simulink model "ecan2essai"  (Simulink 7.0)
settings: Solver=FixedStepDiscrete  StartTime=0.0  StopTime=10.0  FixedStep=0.001  RelTol=1e-3
undefined symbols (not defined in the file or in its folder): Configuration, Initialization, QEIInit, u1, u2, u3
libraries: dsPICdrivers x12, simulink x6
settings Model: Creator=Administrator  LastModifiedBy=Administrator
settings OptimizationCC: OptimizeModelRefInitCode=on  LifeSpan=1
settings DebuggingCC: SignalResolutionControl=TryResolveAllWithWarning
settings HardwareCC: ProdBitPerInt=16  ProdEndianess=LittleEndian  ProdWordSize=16  ProdHWDeviceType=16-bit Generic  TargetHWDeviceType=32-bit Generic
settings RTWCC: SystemTargetFile=dspic.tlc  TemplateMakefile=dspic_pic30_gcc.tmf  PostCodeGenCommand=dsPIC_Compile()  Description=Embedded Target for Microchip dsPIC (real-time)  GenerateReport=on  ProcessScript=dspic_make_rtw_hook  IncludeHyperlinkInReport=on  LaunchReport=on
settings RTWCC: CustomSource=|
  | ecan.c
  | ecan2simulink.c
  | QEI_Functions.c
settings CodeAppCC: IgnoreCustomStorageClasses=off
settings STFCustomTargetCC: GenFloatMathFcnCalls=ANSI_C  ModelReferenceCompliant=off  IncludeMdlTerminateFcn=off  CombineOutputUpdateFcns=on  SuppressErrorStatus=on  ERTCustomFileBanners=on  SupportContinuousTime=off  SupportNonInlinedSFcns=off  SystemTargetFile=dspic.tlc
settings ERTTargetCC: GenFloatMathFcnCalls=ANSI_C  ModelReferenceCompliant=off  CompOptLevelCompliant=off  IncludeMdlTerminateFcn=off  SuppressErrorStatus=on  ModelStepFunctionPrototypeControlCompliant=off  ExtModeMexFile=noextcomm  InlinedParameterPlacement=NonHierarchical  ERTSrcFileBannerTemplate=dsPIC_code_template.cgt  ERTHdrFileBannerTemplate=dsPIC_code_template.cgt  ERTDataSrcFileTemplate=dsPIC_code_template.cgt  ERTDataHdrFileTemplate=dsPIC_code_template.cgt  ERTCustomFileTemplate=dsPIC_main.tlc  ModuleNamingRule=SameAsModel  EnableUserReplacementTypes=on
settings CustomProperty: DataType=string  Value=C:\PROGRA~1\MATLAB\R2007b\bin\win32\gmake

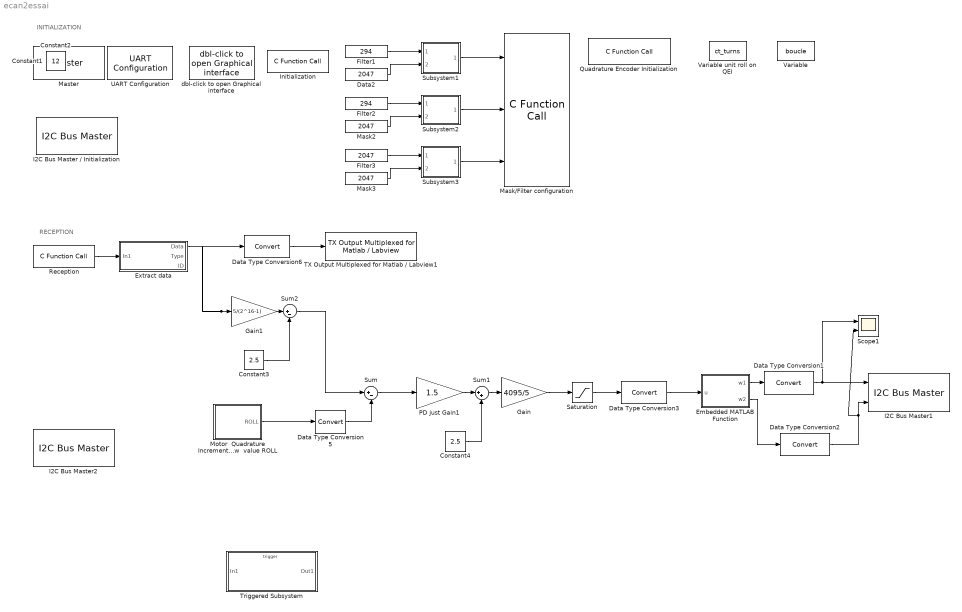
== system ecan2essai ==
  note: RECEPTION
  note: INITIALIZATION
  Constant3 : Constant  Value=2.5  OutDataType=sfix(16)  OutScaling=2^0
  Constant4 : Constant  Value=2.5  OutDataType=sfix(16)  OutScaling=2^0
  Data Type Conversion1 : DataTypeConversion  OutMin=[0]  OutMax=[255]  OutDataTypeMode=uint8  OutDataType=sfix(16)  OutScaling=2^0  ConvertRealWorld=Stored Integer (SI)  RndMeth=Zero
  Data Type Conversion2 : DataTypeConversion  OutMin=[0]  OutMax=[255]  OutDataTypeMode=uint8  OutDataType=sfix(16)  OutScaling=2^0  ConvertRealWorld=Stored Integer (SI)  RndMeth=Zero
  Data Type Conversion3 : DataTypeConversion  OutMin=[0]  OutMax=[4095]  OutDataTypeMode=uint16  OutDataType=sfix(16)  OutScaling=2^0  RndMeth=Zero
  Data Type Conversion5 : DataTypeConversion  OutMin=[0]  OutMax=[4095]  OutDataTypeMode=double  OutDataType=sfix(16)  OutScaling=2^0  RndMeth=Zero
  Data Type Conversion6 : DataTypeConversion  OutMin=[0]  OutMax=[4095]  OutDataTypeMode=uint16  OutDataType=sfix(16)  OutScaling=2^0  RndMeth=Zero
  Data2 : Constant  Value=2047  OutDataTypeMode=uint32  OutDataType=sfix(16)  OutScaling=2^0
  Embedded MATLAB Function : Stateflow chart
  Extract data : Subsystem
  Filter1 : Constant  Value=294  OutDataTypeMode=uint32  OutDataType=sfix(16)  OutScaling=2^0
  Filter2 : Constant  Value=294  OutDataTypeMode=uint32  OutDataType=sfix(16)  OutScaling=2^0
  Filter3 : Constant  Value=2047  OutDataTypeMode=uint32  OutDataType=sfix(16)  OutScaling=2^0
  Gain : Gain  Gain=4095/5  ParameterDataType=sfix(16)  ParameterScaling=2^0  OutDataType=sfix(16)  OutScaling=2^0
  Gain1 : Gain  Gain=5/(2^16-1)  ParameterDataType=sfix(16)  ParameterScaling=2^0  OutDataType=sfix(16)  OutScaling=2^0
  "I2C Bus Master / Initialization " : dsPICdrivers/BUS I2C/I2C Bus Master  Tag=dsPIC_I2C_Master  NumI2C=1  Sequence='S A024 W056 W000 W001 P'  InitializeOnceOnly=When PIC is initialized (only once)  Enable=on  WaitAfterEnable=3  Disable=off  AdressNbrBits=7 bits  I2CBusFreq=363  SlewRate=off  SMBUSThreshold=off  OutputErrorFlag=off  SampleTime=-1  OrderingInOutPopup=None  Info=Fscl = 100 KHz
  I2C Bus Master1 : dsPICdrivers/BUS I2C/I2C Bus Master  Tag=dsPIC_I2C_Master  NumI2C=1  Sequence='S A024 W016 W W P'  InitializeOnceOnly=When I2C bus is enable (if Enable I2C is checked)  Enable=on  WaitAfterEnable=3  Disable=off  AdressNbrBits=7 bits  I2CBusFreq=363  SlewRate=off  SMBUSThreshold=off  OutputErrorFlag=off  SampleTime=-1  OrderingInOutPopup=None  Info=Fscl = 100 KHz
  I2C Bus Master2 : dsPICdrivers/BUS I2C/I2C Bus Master  Tag=dsPIC_I2C_Master  NumI2C=1  Sequence='S A024 W048 W000 W003P'  InitializeOnceOnly=When PIC is initialized (only once)  Enable=on  WaitAfterEnable=3  Disable=off  AdressNbrBits=7 bits  I2CBusFreq=363  SlewRate=off  SMBUSThreshold=off  OutputErrorFlag=off  SampleTime=-1  OrderingInOutPopup=None  Info=Fscl = 100 KHz
  Initialization : dsPICdrivers/OTHERS/C Function Call  Tag=dsPIC_dsPIC_CFunctionCall  fctName='Initialization'  INPUT_SIZE=1  INPUT1=--  INPUT2=--  INPUT3=--  OUTPUT_SIZE=1  OUTPUT1=--  SampleTime=inf  InputType=[ ]  OutputType=[ ]  FctDeclaration=extern void Initialization();  FctCall=Initialization();  OrderingInOutPopup=None
  Mask/Filter configuration : dsPICdrivers/OTHERS/C Function Call  Tag=dsPIC_dsPIC_CFunctionCall  fctName='Configuration'  INPUT_SIZE=1  INPUT1=uint32  INPUT2=uint32  INPUT3=uint32  OUTPUT_SIZE=1  OUTPUT1=--  SampleTime=inf  InputType=[ 6 6 6 ]  OutputType=[ ]  FctDeclaration=extern void Configuration(uint32_T u1, uint32_T u2, uint32_T u3);  FctCall=Configuration(%u1, %u2, %u3);  OrderingInOutPopup=None
  Mask2 : Constant  Value=2047  OutDataTypeMode=uint32  OutDataType=sfix(16)  OutScaling=2^0
  Mask3 : Constant  Value=2047  OutDataTypeMode=uint32  OutDataType=sfix(16)  OutScaling=2^0
  Master : dsPICdrivers/Master  Tag=dsPIC_MASTER  Priority=1  TimeStepType=Timer1  picType=33fJ256MC710  fcy=40000000  Quartz_33f=8e6  PLLActive_33f=on  fcyDesired_33f=40000000  tmr1="[1  39999  0]"  tmr1Info="Time Step : 0.001  ;   Error : 0%  PR1=39999"  tmr2345="[0  0  0  0  0  0  0  0]"  tmr2345cfg=[-1 -1 -1 -1 -1 -1 -1 -1]  IOautoConf=on  typePort="[ 0   0   0   0   0   0   0   0   0   0   0   0   0   0   0   0   0   0   0   0   0   0   0   0   0   0   0   0   0   0   0   0   0   0   0   0   0   0   0   0   0   0   0   0   0   0   0   0   0   0   0   0   0   0   0   0   0   0   0   0   0   0   0   0   0   0   0   0   0   0   0   0   0   0   0   0   0   0   0   0   0   0   0   0   4   5   0   0   0   0   0   0   0   0   0   0   0   0  20  20   0   0   0   0   0   0   0   0   0   0   0   0 ]"  TRIS="[ 65535  65535  65535  65535  65535  65535  65535 ]"  ADPCFG=0  MasterBusyPort=None  MasterOverloadPort=None  FOSC=Quartz (XT - HS)  ClockSwitchMonitor=Both disabled  TempProtection_33f=TEMP_ON  FPBOR=<empty>  PWRT=disable  MCLR=<empty>  PowerSave=off  OverrideFcy=off  NewFcy=1e6  PR2345="[65535  65535  65535  65535  65535  65535  65535  65535]"
  Motor  Quadrature Incremental Encoder  to screw  value ROLL : Subsystem
  PD just Gain1 : Gain  Gain=1.5  ParameterDataType=sfix(16)  ParameterScaling=2^0  OutDataType=sfix(16)  OutScaling=2^0
  Quadrature Encoder Initialization : dsPICdrivers/OTHERS/C Function Call  Tag=dsPIC_dsPIC_CFunctionCall  fctName='QEIInit'  INPUT_SIZE=1  INPUT1=--  INPUT2=--  INPUT3=--  OUTPUT_SIZE=1  OUTPUT1=--  SampleTime=inf  InputType=[ ]  OutputType=[ ]  FctDeclaration=extern void QEIInit();  FctCall=QEIInit();  OrderingInOutPopup=None
  Reception : dsPICdrivers/OTHERS/C Function Call  Tag=dsPIC_dsPIC_CFunctionCall  fctName='Reception'  INPUT_SIZE=1  INPUT1=--  INPUT2=--  INPUT3=--  OUTPUT_SIZE=1  OUTPUT1=uint32  SampleTime=0.001  InputType=[ ]  OutputType=[ 6 ]  FctDeclaration=extern uint32_T Reception();  FctCall=%y1 = Reception();  OrderingInOutPopup=None
  Saturation : Saturate  UpperLimit=4095  LowerLimit=0  OutDataType=sfix(16)  OutScaling=2^0
  Scope1 : Scope  NumInputPorts=2
      settings: YMin=-5~-5  YMax=5~5  MaxDataPoints=50000  SampleInput=on
  Subsystem1 : Subsystem
  Subsystem2 : Subsystem
  Subsystem3 : Subsystem
  Sum : Sum  Inputs=|+-  OutDataTypeMode=double  OutDataType=sfix(16)  OutScaling=2^0
  Sum1 : Sum  Inputs=|++  OutDataTypeMode=double  OutDataType=sfix(16)  OutScaling=2^0
  Sum2 : Sum  Inputs=|+-  OutDataTypeMode=double  OutDataType=sfix(16)  OutScaling=2^0
  TX Output Multiplexed for Matlab / Labview1 : dsPICdrivers/Serial PORT/TX Output Multiplexed for Matlab // Labview  Tag=dsPIC_TX_Multiplexed  Priority=5  UART=2  CleverSpreadingChk=on  CleverSpreading=1  CHANNEL=[0]  CHANNELBLOCKED=[]  CHANNELBLOCKED_BITEWISE=0  Status=OK
  Triggered Subsystem : Subsystem  TreatAsAtomicUnit=on
  UART Configuration : dsPICdrivers/Serial PORT/UART Configuration  Tag=dsPIC_config_UART  Priority=2  UART=2  proposed_BAUD=115200  ALT_TX_RX=on  InterruptTxWhen=When Transmit Buffer is empty  TXInterruptPri=1  TxBufferSize=32  TXEN=on  InterruptRxWhen=When Receive Buffer is full (contain 4 characters)  RXInterruptPri=2  RxBufferSize=32  BAUD=115200  UxBRG=21  Info="UxBRG = 21   ||  Real Baud : 113636   ||  % error : -1.3573  ||  max 11.3636 Bytes / Step"  RealBaud=0
  Variable : DataStoreMemory  DataStoreName=boucle  ReadBeforeWriteMsg=warning  WriteAfterWriteMsg=warning  WriteAfterReadMsg=warning  DataType=uint8  OutDataType=sfix(16)  OutScaling=2^0
      settings: RTWStateStorageClass=ExportedGlobal
  Variable unit roll on QEI : DataStoreMemory  DataStoreName=ct_turns  ReadBeforeWriteMsg=warning  WriteAfterWriteMsg=warning  WriteAfterReadMsg=warning  DataType=int16  OutDataType=sfix(16)  OutScaling=2^0
      settings: RTWStateStorageClass=ExportedGlobal
  dbl-click to open Graphical interface : dsPICdrivers/Serial PORT/dbl-click to open Graphical interface  SystemSampleTime=-1  Nothing=0
  Constant1 : Constant  IOType=siggen  OutDataType=sfix(16)  OutScaling=2^0
  Constant2 : Constant  IOType=siggen  Value=12  OutDataTypeMode=uint32  OutDataType=sfix(16)  OutScaling=2^0
  wires:
  Reception/1 -> Extract data/1(In1)
  Subsystem1/1(Out1) -> Mask/Filter configuration/1
  Filter1/1 -> Subsystem1/1(Filter)
  Data2/1 -> Subsystem1/2(Mask)
  Subsystem2/1(Out1) -> Mask/Filter configuration/2
  Subsystem3/1(Out1) -> Mask/Filter configuration/3
  Filter2/1 -> Subsystem2/1(Filter)
  Mask2/1 -> Subsystem2/2(Mask)
  Filter3/1 -> Subsystem3/1(Filter)
  Mask3/1 -> Subsystem3/2(Mask)
  Extract data/1(Data) -> Gain1/1, Data Type Conversion6/1
  Embedded MATLAB Function/1(w1) -> Data Type Conversion1/1
  Data Type Conversion1/1 -> Scope1/1, I2C Bus Master1/1
  Embedded MATLAB Function/2(w2) -> Data Type Conversion2/1
  Data Type Conversion2/1 -> Scope1/2, I2C Bus Master1/2
  Motor  Quadrature Incremental Encoder  to screw  value ROLL/1(ROLL) -> Data Type Conversion5/1
  Data Type Conversion3/1 -> Embedded MATLAB Function/1(u)
  Data Type Conversion5/1 -> Sum/2
  Sum1/1 -> Gain/1
  PD just Gain1/1 -> Sum1/1
  Constant4/1 -> Sum1/2
  Saturation/1 -> Data Type Conversion3/1
  Data Type Conversion6/1 -> TX Output Multiplexed for Matlab / Labview1/1
  Gain/1 -> Saturation/1
  Sum/1 -> PD just Gain1/1
  Gain1/1 -> Sum2/1
  Constant3/1 -> Sum2/2
  Sum2/1 -> Sum/1

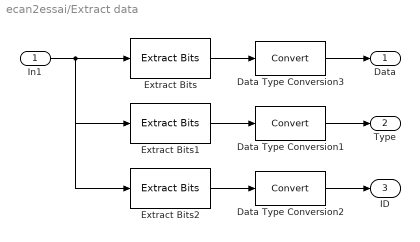
== system ecan2essai/Extract data ==
  In1 : Inport  OutDataType=sfix(16)  OutScaling=2^0
  Data Type Conversion1 : DataTypeConversion  OutMin=[0]  OutMax=[255]  OutDataTypeMode=uint8  OutDataType=sfix(16)  OutScaling=2^0  RndMeth=Zero
  Data Type Conversion2 : DataTypeConversion  OutMin=[0]  OutMax=[1024]  OutDataTypeMode=uint16  OutDataType=sfix(16)  OutScaling=2^0  RndMeth=Zero
  Data Type Conversion3 : DataTypeConversion  OutMin=[0]  OutMax=[1024]  OutDataTypeMode=uint16  OutDataType=sfix(16)  OutScaling=2^0  RndMeth=Zero
  Extract Bits : simulink/Logic and Bit Operations/Extract Bits  SystemSampleTime=-1  bitsToExtract=Upper half  numBits=8  bitIdxRange=[0 7]  outScalingMode=Treat bit field as an integer
  Extract Bits1 : simulink/Logic and Bit Operations/Extract Bits  SystemSampleTime=-1  bitsToExtract=Range of bits  numBits=8  bitIdxRange=[12 15]  outScalingMode=Treat bit field as an integer
  Extract Bits2 : simulink/Logic and Bit Operations/Extract Bits  SystemSampleTime=-1  bitsToExtract=Range of bits  numBits=8  bitIdxRange=[0 11]  outScalingMode=Treat bit field as an integer
  Data : Outport  OutDataType=sfix(16)  OutScaling=2^0
  Type : Outport  Port=2  OutDataType=sfix(16)  OutScaling=2^0
  ID : Outport  Port=3  OutDataType=sfix(16)  OutScaling=2^0
  wires:
  In1/1 -> Extract Bits/1, Extract Bits1/1, Extract Bits2/1
  Extract Bits/1 -> Data Type Conversion3/1
  Extract Bits1/1 -> Data Type Conversion1/1
  Extract Bits2/1 -> Data Type Conversion2/1
  Data Type Conversion2/1 -> ID/1
  Data Type Conversion1/1 -> Type/1
  Data Type Conversion3/1 -> Data/1

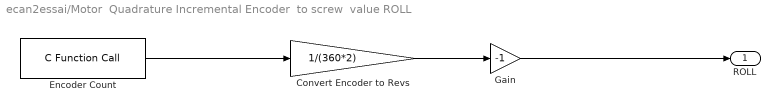
== system ecan2essai/Motor  Quadrature Incremental Encoder  to screw  value ROLL ==
  Convert Encoder to Revs : Gain  Gain=1/(360*2)  ParameterDataType=sfix(16)  ParameterScaling=2^0  OutDataType=sfix(16)  OutScaling=2^0
  Encoder Count : dsPICdrivers/OTHERS/C Function Call  Tag=dsPIC_dsPIC_CFunctionCall  fctName='GetQEI'  INPUT_SIZE=1  INPUT1=--  INPUT2=--  INPUT3=--  OUTPUT_SIZE=1  OUTPUT1=real32  SampleTime=.001  InputType=[ ]  OutputType=[ 7 ]  FctDeclaration=extern real32_T GetQEI();  FctCall=%y1 = GetQEI();  OrderingInOutPopup=None
  Gain : Gain  Gain=-1  ParameterDataType=sfix(16)  ParameterScaling=2^0  OutDataType=sfix(16)  OutScaling=2^0
  ROLL : Outport  OutDataType=sfix(16)  OutScaling=2^0
  wires:
  Encoder Count/1 -> Convert Encoder to Revs/1
  Convert Encoder to Revs/1 -> Gain/1
  Gain/1 -> ROLL/1

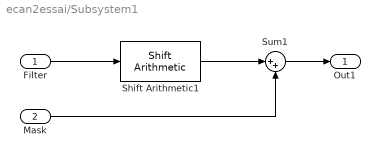
== system ecan2essai/Subsystem1 ==
  Filter : Inport  OutDataType=sfix(16)  OutScaling=2^0
  Mask : Inport  Port=2  OutDataType=sfix(16)  OutScaling=2^0
  Shift Arithmetic1 : simulink/Logic and Bit Operations/Shift Arithmetic  SystemSampleTime=-1  nBitShiftRight=-16  nBinPtShiftRight=0
  Sum1 : Sum  Inputs=|++  OutDataType=sfix(16)  OutScaling=2^0
  Out1 : Outport  OutDataType=sfix(16)  OutScaling=2^0
  wires:
  Sum1/1 -> Out1/1
  Mask/1 -> Sum1/2
  Filter/1 -> Shift Arithmetic1/1
  Shift Arithmetic1/1 -> Sum1/1

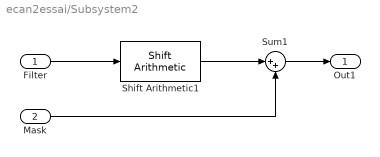
== system ecan2essai/Subsystem2 ==
  Filter : Inport  OutDataType=sfix(16)  OutScaling=2^0
  Mask : Inport  Port=2  OutDataType=sfix(16)  OutScaling=2^0
  Shift Arithmetic1 : simulink/Logic and Bit Operations/Shift Arithmetic  SystemSampleTime=-1  nBitShiftRight=-16  nBinPtShiftRight=0
  Sum1 : Sum  Inputs=|++  OutDataType=sfix(16)  OutScaling=2^0
  Out1 : Outport  OutDataType=sfix(16)  OutScaling=2^0
  wires:
  Shift Arithmetic1/1 -> Sum1/1
  Filter/1 -> Shift Arithmetic1/1
  Mask/1 -> Sum1/2
  Sum1/1 -> Out1/1

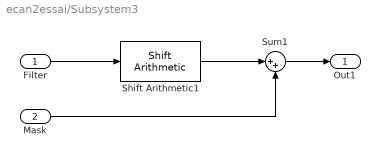
== system ecan2essai/Subsystem3 ==
  Filter : Inport  OutDataType=sfix(16)  OutScaling=2^0
  Mask : Inport  Port=2  OutDataType=sfix(16)  OutScaling=2^0
  Shift Arithmetic1 : simulink/Logic and Bit Operations/Shift Arithmetic  SystemSampleTime=-1  nBitShiftRight=-16  nBinPtShiftRight=0
  Sum1 : Sum  Inputs=|++  OutDataType=sfix(16)  OutScaling=2^0
  Out1 : Outport  OutDataType=sfix(16)  OutScaling=2^0
  wires:
  Sum1/1 -> Out1/1
  Mask/1 -> Sum1/2
  Filter/1 -> Shift Arithmetic1/1
  Shift Arithmetic1/1 -> Sum1/1

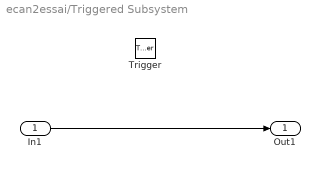
== system ecan2essai/Triggered Subsystem ==
  In1 : Inport  OutDataType=sfix(16)  OutScaling=2^0
  Trigger : TriggerPort
  Out1 : Outport  OutDataType=sfix(16)  OutScaling=2^0
  wires:
  In1/1 -> Out1/1

== matlab function Embedded MATLAB Function ==
  data: u input inherited; w1 output inherited; w2 output inherited
function [w1,w2] = fcn(u)

% Funktion to send the right value to the I²C block
% input: u, a signal from 0 - 4095 
% output:   w1 for the MSB
%           w2 for the LSB 




w2_1 = bitshift(u,12,16);

w2 = bitshift(w2_1,-8,16);


w1 = bitshift(u,-4,16);

end
